simulink model "model6_onoff"  (R2024a)
settings: Solver=VariableStepAuto  StartTime=0.0  StopTime=8760  RelTol=1e-3
model workspace (MAT data in the model file):
  agentObj = 67
undefined symbols (not defined in the file): bat_deseado, bat_inicial, dia_radiacion, dia_solar, difh, dni, ghi, glb, sun_vector, viento
libraries: simulink x1
settings Model: Creator=danie  LastModifiedBy=danie
settings SolverCC: ZeroCrossAlgorithm=Adaptive
settings DebuggingCC: IgnoredZcDiagnostic=none

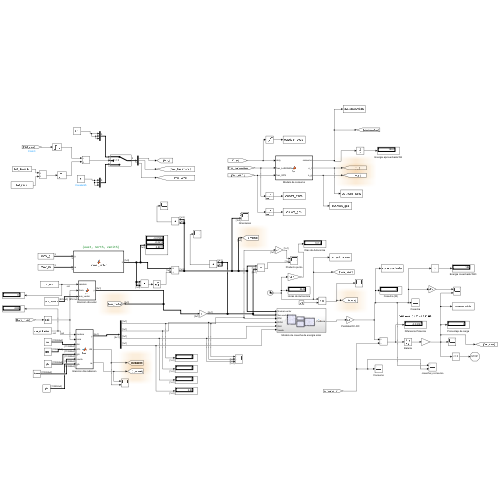
[thumbnail: Simulink's stored preview of the top-level diagram]
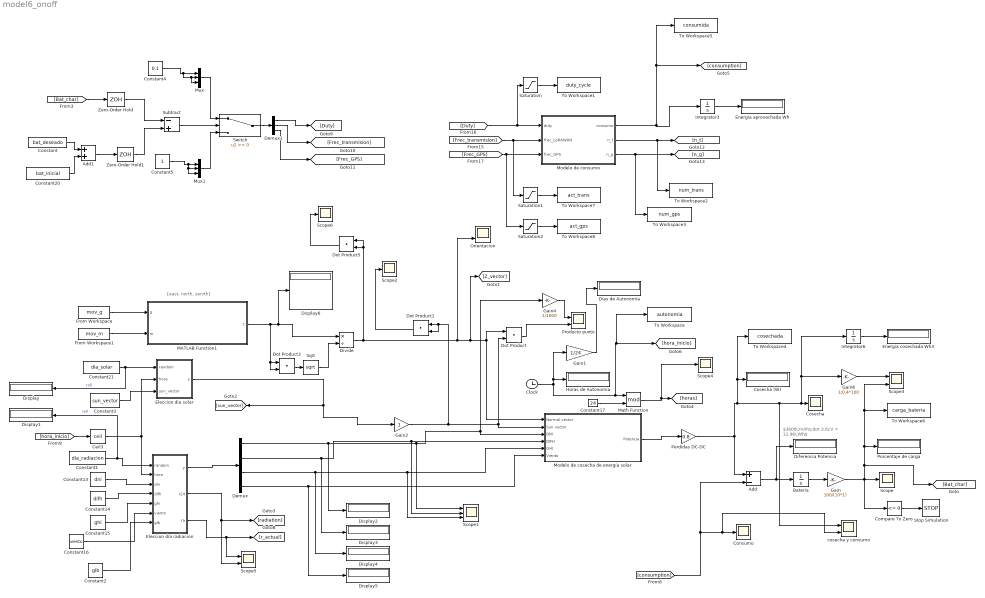
== system model6_onoff ==
  note: $3600\:mAh\cdot 3.6\:V = 12.96\:Wh$
  note: {east, north, zenith}
  Add : Sum  Inputs=+-
  Add1 : Sum
  Batería : Integrator  InitialCondition=10*1*(bat_inicial/100)  LimitOutput=on  UpperSaturationLimit=10*1  LowerSaturationLimit=0
  Ceil3 : Rounding  Operator=ceil
  Clock : Clock
  Compare To Zero : simulink/Logic and Bit Operations/Compare To Zero  relop=<=  OutDataTypeStr=boolean
  Constant : Constant  Value=bat_deseado
  Constant1 : Constant  Value=dia_radiacion
  Constant13 : Constant  Value=dni
  Constant14 : Constant  Value=difh
  Constant15 : Constant  Value=ghi
  Constant16 : Constant  Value=viento
  Constant17 : Constant  Value=24
  Constant2 : Constant  Value=glb
  Constant20 : Constant  Value=bat_inicial
  Constant21 : Constant  Value=dia_solar
  Constant3 : Constant  Value=sun_vector
  Constant4 : Constant  Value=0.1
  Constant5 : Constant
  Consumo : Scope
  Cosecha : Scope
  Cosecha (W) : Display
  Demux : Demux
  Demux1 : Demux  Outputs=3
  Diferencia Potencia : Display
  Display{,1..6} (7 alike) : Display
  Divide : Product  Inputs=*/
  Dot Product{,1,3,5} (4 alike) : DotProduct  OutDataTypeStr=Inherit: Inherit via internal rule
  Días de Autonomía : Display
  Eleccion día radiacion : MATLAB Function  TreatAsAtomicUnit=on
  Eleccion día solar : MATLAB Function  TreatAsAtomicUnit=on
  Energia aprovechada Wh : Display
      settings: Decimation=5
  Energia cosechada Wh3 : Display
      settings: Decimation=5
  From Workspace : FromWorkspace  VariableName=mov_g  SampleTime=1
  From Workspace1 : FromWorkspace  VariableName=mov_m  SampleTime=1
  Gain : Gain  Gain=100/(10*1)
  Gain1 : Gain  Gain=1/24
  Gain2 : Gain
  Gain4 : Gain  Gain=1/1000
  Gain6 : Gain  Gain=1/0.4*100
  Horas de Autonomía : Display
  Integrator3 : Integrator
  Integrator6 : Integrator
  MATLAB Function1 : MATLAB Function  TreatAsAtomicUnit=on
  Math Function : Math  Operator=mod
  Modelo de consumo : MATLAB Function  TreatAsAtomicUnit=on
  Modelo de cosecha de energía solar : Subsystem
  Mux : Mux  Inputs=3
  Mux1 : Mux  Inputs=3
  Orientacion : Scope  NumInputPorts=2
  Perdidas DC-DC : Gain  Gain=0.8
  Porcentaje de carga : Display
  Producto punto : Scope  NumInputPorts=2
  Saturation : Saturate  UpperLimit=1  LowerLimit=0.1
  Saturation1 : Saturate  UpperLimit=1  LowerLimit=0.1
  Saturation2 : Saturate  UpperLimit=1  LowerLimit=0.1
  Scope{,2,4,6} (4 alike) : Scope
  Scope1 : Scope  NumInputPorts=3
  Scope3 : Scope  NumInputPorts=2
  Scope5 : Scope  NumInputPorts=2
  Sqrt : Sqrt
  Stop Simulation : Stop
  Subtract : Sum  Inputs=-+
  Switch : Switch  SaturateOnIntegerOverflow=off  InputSameDT=off
  To Workspace : ToWorkspace  VariableName=autonomia  SaveFormat=Timeseries  SampleTime=1
  To Workspace1 : ToWorkspace  VariableName=duty_cycle  SaveFormat=Timeseries  SampleTime=1
  To Workspace2 : ToWorkspace  VariableName=num_trans  SaveFormat=Timeseries  SampleTime=1
  To Workspace3 : ToWorkspace  VariableName=num_gps  SaveFormat=Timeseries  SampleTime=1
  To Workspace4 : ToWorkspace  VariableName=cosechada  SaveFormat=Timeseries  SampleTime=1
  To Workspace5 : ToWorkspace  VariableName=consumida  SaveFormat=Timeseries  SampleTime=1
  To Workspace6 : ToWorkspace  VariableName=carga_bateria  SaveFormat=Timeseries  SampleTime=1
  To Workspace7 : ToWorkspace  VariableName=act_trans  SaveFormat=Timeseries  SampleTime=-1
  To Workspace8 : ToWorkspace  VariableName=act_gps  SaveFormat=Timeseries  SampleTime=-1
  Zero-Order Hold : ZeroOrderHold
  Zero-Order Hold1 : ZeroOrderHold
  cosecha y consumo : Scope  NumInputPorts=2
  wires:
  Add/1 -> Diferencia Potencia/1, Batería/1
  Batería/1 -> Gain/1
  Gain/1 -> Compare To Zero/1, [Bat_char], To Workspace6/1, Scope3/2, Porcentaje de carga/1, Scope/1
  [consumption] -> Add/2, cosecha y consumo/2, Consumo/1
  Clock/1 -> To Workspace/1, [hora_inicio], Math Function/1, Gain1/1, Horas de Autonomía/1
  Gain1/1 -> Días de Autonomía/1
  Demux/2 -> Display3/1, Scope1/2, Modelo de cosecha de energía solar/4(DIFH)
  Demux/3 -> Display4/1, Scope1/3, Modelo de cosecha de energía solar/5(GHI)
  Demux/4 -> Display5/1, Modelo de cosecha de energía solar/6(Viento)
  Gain2/1 -> Dot Product1/2, Dot Product1/1, Dot Product/2, Modelo de cosecha de energía solar/2(Sun vector)
  Dot Product/1 -> Producto punto/2
  Dot Product1/1 -> Scope2/1
  Eleccion día solar/1(y) -> Gain2/1, [sun_vector]
  Gain4/1 -> Producto punto/1
  Gain6/1 -> Scope3/1
  Modelo de cosecha de energía solar/1(Potencia) -> Perdidas DC-DC/1
  Dot Product3/1 -> Sqrt/1
  Eleccion día radiacion/1(y) -> Demux/1
  Ceil3/1 -> Eleccion día radiacion/2(hora), Eleccion día solar/2(hora)
  Constant21/1 -> Display/1, Eleccion día solar/1(random)  "roll"
  Constant13/1 -> Eleccion día radiacion/3(dni)
  Constant14/1 -> Eleccion día radiacion/4(difh)
  Constant15/1 -> Eleccion día radiacion/5(ghi)
  Constant16/1 -> Eleccion día radiacion/6(viento)
  Constant3/1 -> Eleccion día solar/3(sun_vector)
  [hora_inicio] -> Ceil3/1
  Eleccion día radiacion/2(r24) -> [radiation], Scope5/2
  Modelo de consumo/1(consumo) -> Integrator3/1, To Workspace5/1, [consumption]
  Math Function/1 -> Scope4/1, [horas]
  Constant17/1 -> Math Function/2
  Integrator3/1 -> Energia aprovechada Wh/1
  Constant/1 -> Add1/1
  Constant20/1 -> Add1/2
  Demux1/1 -> [Duty]
  Demux1/2 -> [Frec_transmision]
  Integrator6/1 -> Energia cosechada Wh3/1
  Perdidas DC-DC/1 -> cosecha y consumo/1, Integrator6/1, Gain6/1, Cosecha/1, To Workspace4/1, Cosecha (W)/1, Add/1
  Sqrt/1 -> Divide/2
  Dot Product5/1 -> Scope6/1
  Divide/1 -> Orientacion/2, [Z_vector], Modelo de cosecha de energía solar/1(Normal vector), Dot Product/1, Dot Product5/1, Dot Product5/2
  [Frec_transmision] -> Modelo de consumo/2(frec_LoRAWAN), Saturation1/1
  [Frec_GPS] -> Saturation2/1, Modelo de consumo/3(frec_GPS)
  [Duty] -> Saturation/1, Modelo de consumo/1(duty)
  Demux1/3 -> [Frec_GPS]
  Modelo de consumo/2(n_t) -> To Workspace2/1, [n_t]
  Modelo de consumo/3(n_g) -> To Workspace3/1, [n_g]
  Eleccion día radiacion/3(ra) -> Scope5/1, [r_actual]
  Demux/1 -> Display2/1, Scope1/1, Gain4/1, Modelo de cosecha de energía solar/3(DNI)
  Constant2/1 -> Eleccion día radiacion/7(glb)
  From Workspace/1 -> MATLAB Function1/1(g)
  From Workspace1/1 -> MATLAB Function1/2(m)
  MATLAB Function1/1(z) -> Dot Product3/2, Dot Product3/1, Display6/1, Divide/1
  Constant1/1 -> Display1/1, Eleccion día radiacion/1(random)  "roll"
  Compare To Zero/1 -> Stop Simulation/1
  Saturation/1 -> To Workspace1/1
  Saturation1/1 -> To Workspace7/1
  Saturation2/1 -> To Workspace8/1
  Subtract/1 -> Switch/2
  Switch/1 -> Demux1/1
  Mux/1 -> Switch/1
  Mux1/1 -> Switch/3
  Constant4/1 -> Mux/3, Mux/2, Mux/1
  Constant5/1 -> Mux1/3, Mux1/2, Mux1/1
  [Bat_char] -> Zero-Order Hold/1
  Zero-Order Hold/1 -> Subtract/1
  Add1/1 -> Zero-Order Hold1/1
  Zero-Order Hold1/1 -> Subtract/2

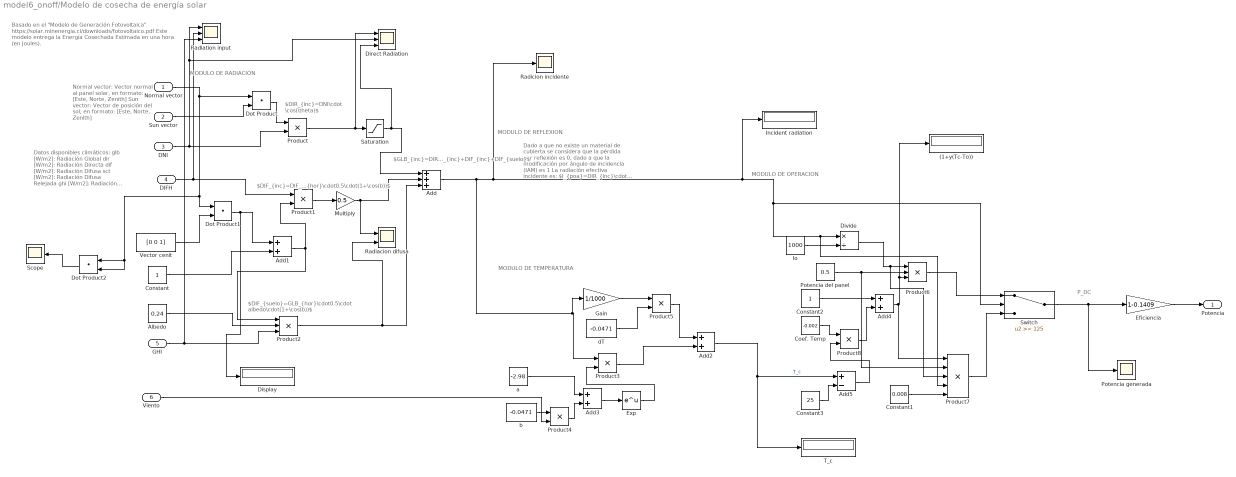
== system model6_onoff/Modelo de cosecha de energía solar ==
  note: MODULO DE OPERACION
  note: MODULO DE TEMPERATURA
  note: $DIF_{suelo}=GLB_{hor}\cdot0.5\cdot albedo\cdot(1+\cos(b))$
  note: P_DC
  note: MODULO DE RADIACIÓN
  note: Dado a que no existe un material de cubierta
      | se considera que la pérdida por reflexión es 0,
      | dado a que la modificación por ángulo de
      | incidencia (IAM) es 1
      |
      | La radiación efectiva incidente es:
      | $I_{poa}=DIR_{inc}\cdot IAM+DIF_{inc}+DIF_{suelo}=GLB_{inc}$
  note: Datos disponibles climáticos:
      | glb [W/m2]: Radiación Global
      | dir [W/m2]: Radiación Directa
      | dif [W/m2]: Radiación Difusa
      | sct [W/m2]: Radiación Difusa Relejada
      | ghi [W/m2]: Radiación Global Horizontal
      | dirh [W/m2]: Radiación Directa
      | difh [W/m2]: Radiación Difusa
      | dni [W/m2]: Radiación Directa Normal
      | temp [C]: Temperatura en 2 metros (correjida)
      | vel [m/s]: Velocidad de Viento
      | shadow [0: sin, 1: con]: Sobra debido a topografía
      | cloud [1: si, 0: no]: Presencia de nubes
  note: MODULO DE REFLEXION
  note: $GLB_{inc}=DIR_{inc}+DIF_{inc}+DIF_{suelo}$
  note: $DIF_{inc}=DIF_{hor}\cdot0.5\cdot(1+\cos(b))$
  note: Basado en el "Modelo de Generación Fotovoltaica"
      | https://solar.minenergia.cl/downloads/fotovoltaico.pdf
      |
      | Este modelo entrega la Energía Cosechada Estimada en
      | una hora (en Joules).
  note: $DIR_{inc}=DNI\cdot \cos(\theta)$
  note: Normal vector:
      | Vector normal al panel solar, en formato:
      | [Este, Norte, Zenith]
      |
      | Sun vector:
      | Vector de posición del sol, en formato:
      | [Este, Norte, Zenith]
  Normal vector : Inport  PortDimensions=3
  Sun vector : Inport  Port=2  PortDimensions=3
  DNI : Inport  Port=3  PortDimensions=1
  DIFH : Inport  Port=4  PortDimensions=1
  GHI : Inport  Port=5  PortDimensions=1
  Viento : Inport  Port=6  PortDimensions=1
  (1+y(Tc-To)) : Display
  Add : Sum  Inputs=+++
  Add{1..4} (4 alike) : Sum
  Add5 : Sum  Inputs=+-
  Albedo : Constant  Value=0.24
  Coef. Temp : Constant  Value=-0.002
  Constant : Constant
  Constant1 : Constant  Value=0.008
  Constant2 : Constant
  Constant3 : Constant  Value=25
  Direct Radiation : Scope  NumInputPorts=3
  Display : Display
  Divide : Product  Inputs=*/
  Dot Product : DotProduct  OutDataTypeStr=Inherit: Inherit via internal rule
  Dot Product1 : DotProduct  OutDataTypeStr=Inherit: Inherit via internal rule
  Dot Product2 : DotProduct  OutDataTypeStr=Inherit: Inherit via internal rule
  Eficiencia : Gain  Gain=1-0.1409
  Exp : Math
  Gain : Gain  Gain=1/1000
  Incident radiation : Display
  Io : Constant  Value=1000
  Multiply : Gain  Gain=0.5
  Potencia del panel : Constant  Value=0.5
  Potencia generada : Scope
  Product{,1,3..5,8} (6 alike) : Product
  Product2 : Product  Inputs=3
  Product6 : Product  Inputs=3
  Product7 : Product  Inputs=5
  Radiacion difusa : Scope  NumInputPorts=2
  Radiation input : Scope  NumInputPorts=3
  Radicion incidente : Scope
  Saturation : Saturate  UpperLimit=Inf
  Scope : Scope
  Switch : Switch  Threshold=125  SaturateOnIntegerOverflow=off  InputSameDT=off
  T_c : Display
  Vector cenit : Constant  Value=[0 0 1]
  a : Constant  Value=-2.98
  b : Constant  Value=-0.0471
  dT : Constant  Value=-0.0471
  Potencia : Outport
  wires:
  Coef. Temp/1 -> Product8/1
  Add2/1 -> T_c/1, Add5/1  "T_c"
  Add3/1 -> Exp/1
  GHI/1 -> Product2/3, Radiation input/3
  Io/1 -> Divide/2
  Constant2/1 -> Add4/1
  Multiply/1 -> Radiacion difusa/1, Add/2
  Product7/1 -> Switch/3
  Product5/1 -> Add2/1
  Product8/1 -> Add4/2
  Divide/1 -> Product7/3, Product6/1
  Constant1/1 -> Product7/5
  Potencia del panel/1 -> Product7/2, Product6/2
  Eficiencia/1 -> Potencia/1
  Gain/1 -> Product5/1
  Add4/1 -> Product7/1, (1+y(Tc-To))/1, Product6/3
  dT/1 -> Product5/2
  a/1 -> Add3/1
  Albedo/1 -> Product2/2
  Viento/1 -> Product4/2
  Exp/1 -> Product3/2
  Add/1 -> Gain/1, Product3/1, Radicion incidente/1, Incident radiation/1, Switch/2, Product7/4, Divide/1
  Switch/1 -> Potencia generada/1, Eficiencia/1
  DIFH/1 -> Radiation input/2, Product1/1
  Product6/1 -> Switch/1
  Add5/1 -> Product8/2
  Product3/1 -> Add2/2
  Sun vector/1 -> Dot Product/2
  Vector cenit/1 -> Dot Product1/2
  Product4/1 -> Add3/2
  b/1 -> Product4/1
  Constant3/1 -> Add5/2
  DNI/1 -> Product/2, Direct Radiation/2, Radiation input/1
  Product2/1 -> Radiacion difusa/2, Add/3
  Constant/1 -> Add1/2
  Normal vector/1 -> Dot Product2/2, Dot Product2/1, Dot Product1/1, Dot Product/1
  Product/1 -> Saturation/1, Direct Radiation/1
  Dot Product1/1 -> Display/1, Add1/1
  Dot Product/1 -> Product/1
  Add1/1 -> Product2/1, Product1/2
  Product1/1 -> Multiply/1
  Saturation/1 -> Direct Radiation/3, Add/1
  Dot Product2/1 -> Scope/1

== matlab function model6_onoff/Eleccion día solar ==
  data: random input; y output; hora input; sun_vector input
function y = fcn(random,hora,sun_vector)

y = zeros(3, 1);
hora = fix(hora);

n_inicial = (random-1)*24 + 1;

y(1) = sun_vector(n_inicial+hora,1);
y(2) = sun_vector(n_inicial+hora,2);
y(3) = sun_vector(n_inicial+hora,3);

== matlab function model6_onoff/Eleccion día radiacion ==
  data: random input; y output; hora input; dni input; difh input; ghi input; viento input; r24 output; ra output; glb input
function [y,r24,ra] = fcn(random,hora,dni,difh,ghi,viento,glb)

y = zeros(4, 1);
hora = fix(hora);
%r24 = zeros(24,1);

r24 = 0;

n_inicial = (random - 1)*24 + 1;
%n_final = n_inicial+24;

y(1) = dni(n_inicial+hora,2);
y(2) = difh(n_inicial+hora,2);
y(3) = ghi(n_inicial+hora,2);
y(4) = viento(n_inicial+hora,2);
ra = glb(n_inicial+hora,2);

for k = 0:23
    r24 = r24 + glb(n_inicial+k,2);
end

r24 = r24/24;


% y(1) = dni;
% y(2) = difh;
% y(3) = ghi;
% y(4) = viento;

== matlab function model6_onoff/Modelo de consumo ==
  data: duty input; consumo output; frec_LoRAWAN input; frec_GPS input; n_t output; n_g output
function [consumo,n_t,n_g]= fcn(duty,frec_LoRAWAN,frec_GPS)

%Salida entre 0.1 y 1

if frec_LoRAWAN >= 1
    n_t = 10;
elseif frec_LoRAWAN >= 0.1
    n_t = fix(frec_LoRAWAN*10);
else
    n_t = 1;
end

if frec_GPS >= 1
    n_g = 10;
elseif frec_GPS >= 0.1
    n_g = fix(frec_GPS*10);
else
    n_g = 1;
end

if duty >= 1
    d = 1;
elseif duty >= 0.1
    d = duty;
else
    d = 0.1;
end

act = 0.097; %Consumo IMU activa
no_act = 0.023; %Consumo IMU no activa
tran = 0.197*1.133/3600; %Consumo de transmisión
GPS = 0.437*48.520/3600; %Consumo de GPS

consumo = act*d + no_act*(1-d) + tran*n_t + GPS*n_g + 19*0.167*5.245/3600;

== matlab function model6_onoff/MATLAB Function1 ==
  data: g input; z output; m input
function z = normal_vector(g,m)
%NORMAL_VECTOR Summary of this function goes here
% Por Daniel Iglesias 2024

%{x y z}
% g = [gx gy gz];
% m = [mx my mz];

%magnitud de los vectores
m_m = (m(1)^2+m(2)^2+m(3)^2)^(1/2);
m_g = (g(1)^2+g(2)^2+g(3)^2)^(1/2);

%coeficientes
A = m(1)/m_m;
B = m(2)/m_m;
C = m(3)/m_m;
D = -g(1)/m_g;
E = -g(2)/m_g;
F = -g(3)/m_g;
G = (m(3)*g(2)-m(2)*g(3))/(m_g*m_m);
H = (m(1)*g(3)-m(3)*g(1))/(m_g*m_m);
I = (m(2)*g(1)-m(1)*g(2))/(m_g*m_m);

div = (A*E*I+B*F*G+C*D*H)-(G*E*C+H*F*A+I*D*B);

% vector normal {east, north, zenith}
z = [(A*E-D*B), (D*H-G*E), (B*G-H*A)]/div;

% opuesto al vector normal
%z_p = -z

end
